simulink model "ProjectACC"  (R2021a)
settings: Solver=FixedStepDiscrete  StartTime=0.0  StopTime=10  FixedStep=0.01  RelTol=1e-3
settings Model: DataDictionary=ProjectACC.sldd  EnableAccessToBaseWorkspace=off  Creator=rajes  LastModifiedBy=rajes
settings OptimizationCC: DefaultParameterBehavior=Inlined  EnhancedBackFolding=on  PassReuseOutputArgsAs=Individual arguments  ZeroExternalMemoryAtStartup=off  ZeroInternalMemoryAtStartup=off  OptimizeBlockOrder=speed  DifferentSizesBufferReuse=on  OptimizationCustomize=off  EfficientTunableParamExpr=on
settings DebuggingCC: SignalInfNanChecking=error  CheckMatrixSingularityMsg=error  IntegerOverflowMsg=error  ParameterTunabilityLossMsg=error  UniqueDataStoreMsg=warning  StrictBusMsg=ErrorOnBusTreatedAsVector  IntegerSaturationMsg=error
settings SFSimCC: MATLABDynamicMemAlloc=off
settings RTWCC: SystemTargetFile=ert.tlc  GenCodeOnly=on  TemplateMakefile=ert_default_tmf
settings CodeAppCC: ForceParamTrailComments=on  IgnoreCustomStorageClasses=off  OperatorAnnotations=on  SimulinkDataObjDesc=on  SFDataObjDesc=on  InsertBlockDesc=on
settings ERTTargetCC: TargetLangStandard=C99 (ISO)  GenerateSampleERTMain=on  InlinedParameterPlacement=NonHierarchical  ERTCustomFileTemplate=example_file_process.tlc

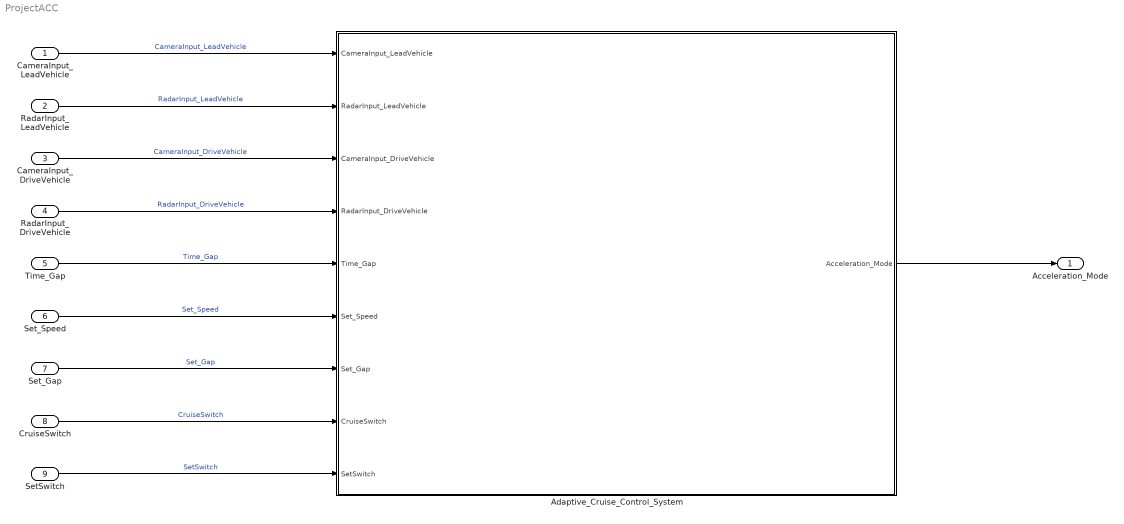
== system ProjectACC ==
  CameraInput_LeadVehicle : Inport
  RadarInput_LeadVehicle : Inport  Port=2
  CameraInput_DriveVehicle : Inport  Port=3
  RadarInput_DriveVehicle : Inport  Port=4
  Time_Gap : Inport  Port=5
  Set_Speed : Inport  Port=6
  Set_Gap : Inport  Port=7
  CruiseSwitch : Inport  Port=8
  SetSwitch : Inport  Port=9
  Adaptive_Cruise_Control_System : Subsystem
  Acceleration_Mode : Outport
  wires:
  CameraInput_LeadVehicle/1 -> Adaptive_Cruise_Control_System/1(CameraInput_LeadVehicle)  "CameraInput_LeadVehicle"
  RadarInput_LeadVehicle/1 -> Adaptive_Cruise_Control_System/2(RadarInput_LeadVehicle)  "RadarInput_LeadVehicle"
  CameraInput_DriveVehicle/1 -> Adaptive_Cruise_Control_System/3(CameraInput_DriveVehicle)  "CameraInput_DriveVehicle"
  RadarInput_DriveVehicle/1 -> Adaptive_Cruise_Control_System/4(RadarInput_DriveVehicle)  "RadarInput_DriveVehicle"
  Time_Gap/1 -> Adaptive_Cruise_Control_System/5(Time_Gap)  "Time_Gap"
  Set_Speed/1 -> Adaptive_Cruise_Control_System/6(Set_Speed)  "Set_Speed"
  Set_Gap/1 -> Adaptive_Cruise_Control_System/7(Set_Gap)  "Set_Gap"
  CruiseSwitch/1 -> Adaptive_Cruise_Control_System/8(CruiseSwitch)  "CruiseSwitch"
  SetSwitch/1 -> Adaptive_Cruise_Control_System/9(SetSwitch)  "SetSwitch"
  Adaptive_Cruise_Control_System/1(Acceleration_Mode) -> Acceleration_Mode/1

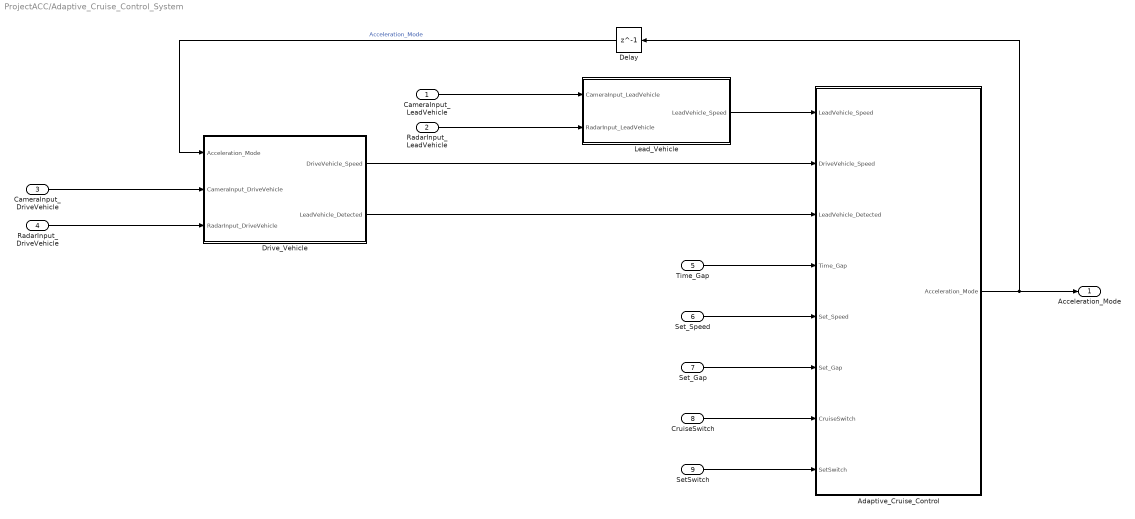
== system ProjectACC/Adaptive_Cruise_Control_System ==
  CameraInput_LeadVehicle : Inport
  RadarInput_LeadVehicle : Inport  Port=2
  CameraInput_DriveVehicle : Inport  Port=3
  RadarInput_DriveVehicle : Inport  Port=4
  Time_Gap : Inport  Port=5
  Set_Speed : Inport  Port=6
  Set_Gap : Inport  Port=7
  CruiseSwitch : Inport  Port=8
  SetSwitch : Inport  Port=9
  Adaptive_Cruise_Control : Stateflow chart  TreatAsAtomicUnit=on
  Delay : Delay  DelayLength=1
  Drive_Vehicle : Subsystem
  Lead_Vehicle : Subsystem
  Acceleration_Mode : Outport
  wires:
  Adaptive_Cruise_Control/1(Acceleration_Mode) -> Acceleration_Mode/1, Delay/1
  Drive_Vehicle/1(DriveVehicle_Speed) -> Adaptive_Cruise_Control/2(DriveVehicle_Speed)
  CruiseSwitch/1 -> Adaptive_Cruise_Control/7(CruiseSwitch)
  Delay/1 -> Drive_Vehicle/1(Acceleration_Mode)  "Acceleration_Mode"
  CameraInput_DriveVehicle/1 -> Drive_Vehicle/2(CameraInput_DriveVehicle)
  Set_Speed/1 -> Adaptive_Cruise_Control/5(Set_Speed)
  CameraInput_LeadVehicle/1 -> Lead_Vehicle/1(CameraInput_LeadVehicle)
  RadarInput_LeadVehicle/1 -> Lead_Vehicle/2(RadarInput_LeadVehicle)
  Lead_Vehicle/1(LeadVehicle_Speed) -> Adaptive_Cruise_Control/1(LeadVehicle_Speed)
  RadarInput_DriveVehicle/1 -> Drive_Vehicle/3(RadarInput_DriveVehicle)
  Set_Gap/1 -> Adaptive_Cruise_Control/6(Set_Gap)
  Time_Gap/1 -> Adaptive_Cruise_Control/4(Time_Gap)
  Drive_Vehicle/2(LeadVehicle_Detected) -> Adaptive_Cruise_Control/3(LeadVehicle_Detected)
  SetSwitch/1 -> Adaptive_Cruise_Control/8(SetSwitch)

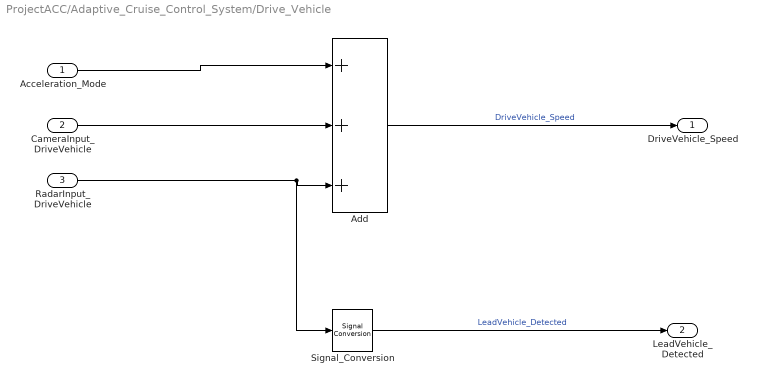
== system ProjectACC/Adaptive_Cruise_Control_System/Drive_Vehicle ==
  Acceleration_Mode : Inport
  CameraInput_DriveVehicle : Inport  Port=2
  RadarInput_DriveVehicle : Inport  Port=3
  Add : Sum  Inputs=+++
  Signal_Conversion : SignalConversion  OverrideOpt=off
  DriveVehicle_Speed : Outport
  LeadVehicle_Detected : Outport  Port=2
  wires:
  Add/1 -> DriveVehicle_Speed/1  "DriveVehicle_Speed"
  Signal_Conversion/1 -> LeadVehicle_Detected/1  "LeadVehicle_Detected"
  RadarInput_DriveVehicle/1 -> Signal_Conversion/1, Add/3
  Acceleration_Mode/1 -> Add/1
  CameraInput_DriveVehicle/1 -> Add/2

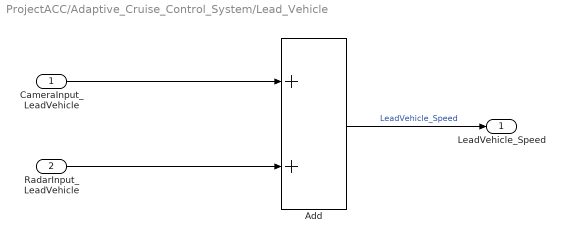
== system ProjectACC/Adaptive_Cruise_Control_System/Lead_Vehicle ==
  CameraInput_LeadVehicle : Inport
  RadarInput_LeadVehicle : Inport  Port=2
  Add : Sum
  LeadVehicle_Speed : Outport
  wires:
  CameraInput_LeadVehicle/1 -> Add/1
  RadarInput_LeadVehicle/1 -> Add/2
  Add/1 -> LeadVehicle_Speed/1  "LeadVehicle_Speed"

== stateflow chart ProjectACC/Adaptive_Cruise_Control_System/Adaptive_Cruise_Control ==
  state ACC_OFFMODE
    en:Acceleration_Mode=0;
  state ACC_STANDBYMODE
    en:Acceleration_Mode=1;
  state ACC_ON_MODE
    en:Acceleration_Mode=0;
    state LeadVehicle_Detected_Follow
      en: Acceleration_Mode=2;
    state LeadVehicle_Detected_Resume
      en:Acceleration_Mode=3;
    state LeadVehicle_Not_Detected_Resume
      en:Acceleration_Mode=1;
    state LeadVehicle_Not_Detected
      en:Acceleration_Mode=1;
    state LeadVehicle_Speed_equal_Set_Speed
      en:Acceleration_Mode=5;
    state LeadVehicle_Speed_Lessthan_Set_Speed
      en:Acceleration_Mode=4;
    (default) -> LeadVehicle_Detected_Follow
    LeadVehicle_Detected_Resume -> LeadVehicle_Detected_Follow [order 1] : [(DriveVehicle_Speed==Set_Speed)&&(LeadVehicle_Speed>=Set_Speed)&&(Time_Gap>=Set_Gap)]
    LeadVehicle_Detected_Resume -> LeadVehicle_Not_Detected_Resume [order 2] : [LeadVehicle_Detected==0]
    LeadVehicle_Not_Detected -> LeadVehicle_Detected_Follow [order 2] : [(LeadVehicle_Detected==1)&&(DriveVehicle_Speed==Set_Speed)&&(LeadVehicle_Speed>=Set_Speed)&&(Time_Gap>=Set_Gap)]
    LeadVehicle_Speed_equal_Set_Speed -> LeadVehicle_Detected_Resume [order 2] : [(DriveVehicle_Speed < Set_Speed) && (LeadVehicle_Speed > DriveVehicle_Speed) || (Time_Gap >= Set_Gap)]
    LeadVehicle_Detected_Resume -> LeadVehicle_Speed_equal_Set_Speed [order 3] : [(DriveVehicle_Speed<Set_Speed)&&(LeadVehicle_Speed>DriveVehicle_Speed)&&(Time_Gap>=Set_Gap)]
    LeadVehicle_Detected_Follow -> LeadVehicle_Not_Detected [order 1] : [LeadVehicle_Detected==0]
    LeadVehicle_Detected_Follow -> LeadVehicle_Speed_Lessthan_Set_Speed [order 2] : [(LeadVehicle_Detected==1)&&(LeadVehicle_Speed<Set_Speed)||(Time_Gap<Set_Gap)]
    LeadVehicle_Speed_equal_Set_Speed -> LeadVehicle_Not_Detected_Resume [order 1] : [(LeadVehicle_Detected == 0) || (DriveVehicle_Speed <= Set_Speed)]
    LeadVehicle_Not_Detected -> LeadVehicle_Speed_Lessthan_Set_Speed [order 1] : [(LeadVehicle_Detected==1)&&(LeadVehicle_Speed<Set_Speed)||(Time_Gap<Set_Gap)]
    LeadVehicle_Speed_Lessthan_Set_Speed -> LeadVehicle_Speed_equal_Set_Speed [order 3] : [(LeadVehicle_Speed<Set_Speed) && (LeadVehicle_Speed<DriveVehicle_Speed) || (Time_Gap == 0.75*Set_Gap)]
    LeadVehicle_Speed_Lessthan_Set_Speed -> LeadVehicle_Not_Detected [order 1] : [(LeadVehicle_Detected==0)&&(DriveVehicle_Speed==Set_Speed)]
    LeadVehicle_Speed_Lessthan_Set_Speed -> LeadVehicle_Speed_equal_Set_Speed [order 2] : [((LeadVehicle_Speed*1.25>=DriveVehicle_Speed) && (LeadVehicle_Speed * 0.75<=DriveVehicle_Speed)) && (DriveVehicle_Speed < Set_Speed) && ((Time_Gap<=1.25*Set_Gap) && (Time_Gap >=0.75*Set_Gap))]
  (default) -> ACC_OFFMODE
  ACC_OFFMODE -> ACC_STANDBYMODE : [CruiseSwitch==1]
  ACC_STANDBYMODE -> ACC_OFFMODE [order 1] : [CruiseSwitch==0]
  ACC_ON_MODE -> ACC_OFFMODE [order 1] : [CruiseSwitch==0]
  ACC_ON_MODE -> ACC_STANDBYMODE [order 2] : [SetSwitch==0]
  ACC_STANDBYMODE -> ACC_ON_MODE [order 2] : [SetSwitch==1]
  data: LeadVehicle_Speed input; DriveVehicle_Speed input; LeadVehicle_Detected input; Time_Gap input; Set_Speed input; Set_Gap input; CruiseSwitch input; SetSwitch input; Acceleration_Mode output
